simulink model "ecu_j1939"  (R2026a)
settings: Solver=FixedStepDiscrete  StopTime=10  FixedStep=0.001  SampleTimeConstraint=STIndependent
Description:
  | J1939 periodic PGN data. Source of truth for firmware/gen/ecu_j1939.
settings Model: Creator=jj1001000  LastModifiedBy=jj1001000
settings OptimizationCC: DefaultUnderspecifiedDataType=single
settings DebuggingCC: ParameterPrecisionLossMsg=none
settings HardwareCC: ProdLargestAtomicInteger=Long  ProdLargestAtomicFloat=Double  ProdHWDeviceType=ARM Compatible->ARM Cortex-M
settings RTWCC: SystemTargetFile=ert.tlc  GenCodeOnly=on  Description=Embedded Coder
settings ERTTargetCC: UtilityFuncGeneration=Shared location  IncludeMdlTerminateFcn=off  CodeInterfacePackaging=Reusable function  SupportNonFinite=off

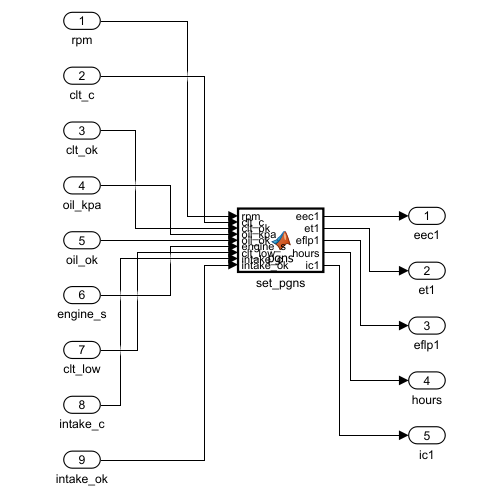
[thumbnail: Simulink's stored preview of the top-level diagram]
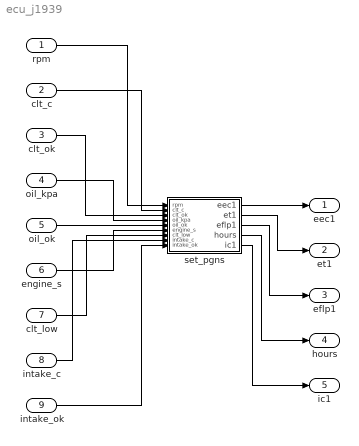
== system ecu_j1939 ==
  rpm : Inport  OutDataTypeStr=single
  clt_c : Inport  Port=2  OutDataTypeStr=single
  clt_ok : Inport  Port=3  OutDataTypeStr=uint8
  oil_kpa : Inport  Port=4  OutDataTypeStr=single
  oil_ok : Inport  Port=5  OutDataTypeStr=uint8
  engine_s : Inport  Port=6  OutDataTypeStr=uint32
  clt_low : Inport  Port=7  OutDataTypeStr=uint8
  intake_c : Inport  Port=8  OutDataTypeStr=single
  intake_ok : Inport  Port=9  OutDataTypeStr=uint8
  set_pgns : MATLAB Function  TreatAsAtomicUnit=on
  eec1 : Outport  OutDataTypeStr=uint8
  et1 : Outport  Port=2  OutDataTypeStr=uint8
  eflp1 : Outport  Port=3  OutDataTypeStr=uint8
  hours : Outport  Port=4  OutDataTypeStr=uint8
  ic1 : Outport  Port=5  OutDataTypeStr=uint8
  wires:
  rpm/1 -> set_pgns/1(rpm)
  clt_c/1 -> set_pgns/2(clt_c)
  clt_ok/1 -> set_pgns/3(clt_ok)
  oil_kpa/1 -> set_pgns/4(oil_kpa)
  oil_ok/1 -> set_pgns/5(oil_ok)
  intake_ok/1 -> set_pgns/9(intake_ok)
  engine_s/1 -> set_pgns/6(engine_s)
  clt_low/1 -> set_pgns/7(clt_low)
  intake_c/1 -> set_pgns/8(intake_c)
  set_pgns/1(eec1) -> eec1/1
  set_pgns/2(et1) -> et1/1
  set_pgns/3(eflp1) -> eflp1/1
  set_pgns/4(hours) -> hours/1
  set_pgns/5(ic1) -> ic1/1

== matlab function ecu_j1939/set_pgns ==
  data: rpm input single; eec1 output uint8; clt_c input single; clt_ok input uint8; oil_kpa input single; oil_ok input uint8; engine_s input uint32; clt_low input uint8; intake_c input single; intake_ok input uint8; et1 output uint8; eflp1 output uint8; hours output uint8; ic1 output uint8
function [eec1, et1, eflp1, hours, ic1] = pgns(rpm, clt_c, clt_ok, oil_kpa, oil_ok, engine_s, clt_low, intake_c, intake_ok)
%#codegen
eec1 = repmat(uint8(255), 8, 1); et1 = eec1; eflp1 = eec1; hours = eec1; ic1 = eec1;
% EEC1: speed, 0.125 rpm/bit, limited to the 8031.875 rpm range
r = rpm;
if r < single(0)
    r = single(0);
elseif r > single(8031)
    r = single(8031);
end
raw = uint16(floor(r / single(0.125) + single(0.5)));
eec1(4) = uint8(bitand(raw, uint16(255)));
eec1(5) = uint8(bitshift(raw, -8));
if clt_ok ~= 0
    et1(1) = byte_clamp(clt_c + single(40));
end
if oil_ok ~= 0
    eflp1(4) = byte_clamp(oil_kpa / single(4));
end
% EFL/P1 byte 8, SPN 111 coolant level, 0.4 %/bit: pin 43 low reads 0 %
if clt_low ~= 0
    eflp1(8) = uint8(0);
else
    eflp1(8) = uint8(250);
end
% IC1 byte 3, SPN 105 intake manifold temperature (pin 79)
if intake_ok ~= 0
    ic1(3) = byte_clamp(intake_c + single(40));
end
% HOURS: 0.05 h = 180 s per bit, little-endian
h = idivide(engine_s, uint32(180));
for i = 1:4
    hours(i) = uint8(bitand(bitshift(h, -8 * (i - 1)), uint32(255)));
end
end

function b = byte_clamp(x)
% 0..250, rounded half up (250 and above are reserved in J1939)
if x < single(0)
    b = uint8(0);
elseif x > single(250)
    b = uint8(250);
else
    b = uint8(floor(x + single(0.5)));
end
end
